simulink model "ACC5v_FFNN_traincgf_30_30_30_ep_50_Nor_20250704"  (R2021a)
settings: Solver=FixedStepAuto  StartTime=0.0  StopTime=T  RelTol=1e-3
undefined symbols (not defined in the file or in its folder): t_gap, Ts, v0_ego, v0_lead, v_set, x0_ego, x0_lead, x_gain, x_offset, y_gain, y_offset
libraries: neural x95
(part 5 of 5)

== system ACC5v_FFNN_traincgf_30_30_30_ep_50_Nor_20250704/Feed-Forward Neural Network/Layer 4/Delays 1 ==
  "p{4}" : Inport  PortDimensions=30
      mask Display: e = 0.06;c1 = [120 230 180]/255;c2 = ([120 230 180]+0)/(256+128);c3 = ([120 230 180]+128)/(256+128);patch([0 1 1 0],[0 0 1 1],c1);patch([0 1 1 1-e 1-e 0+e],[0 0 1 1-e 0+e 0+e],c2);patch([0 0 1 1-e 0+e 0+e],[0 1 1 1-e 1-e 0+e],c3);plot([0 1 1 0 0],[0 0 1 1 0]);
  mux : Mux  Inputs=1
      mask Display: e = 0.06;c1 = [120 150 230]/255;c2 = ([120 150 230]+0)/383;c3 = ([120 150 230]+128)/383;patch([0 1 1 0],[0 0 1 1],c1);patch([0 1 1 1-e 1-e 0+e],[0 0 1 1-e 0+e 0+e],c2);patch([0 0 1 1-e 0+e 0+e],[0 1 1 1-e 1-e 0+e],c3);plot([0 1 1 0 0],[0 0 1 1 0]);disp('Mux')
  "pd{4,3}" : Outport
      mask Display: e = 0.06;c1 = [120 230 180]/255;c2 = ([120 230 180]+0)/(256+128);c3 = ([120 230 180]+128)/(256+128);patch([0 1 1 0],[0 0 1 1],c1);patch([0 1 1 1-e 1-e 0+e],[0 0 1 1-e 0+e 0+e],c2);patch([0 0 1 1-e 0+e 0+e],[0 1 1 1-e 1-e 0+e],c3);plot([0 1 1 0 0],[0 0 1 1 0]);
  wires:
  mux/1 -> "pd{4,3}"/1
  "p{4}"/1 -> mux/1

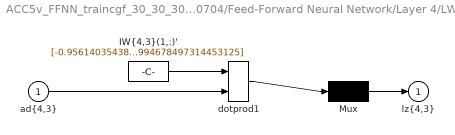
== system ACC5v_FFNN_traincgf_30_30_30_ep_50_Nor_20250704/Feed-Forward Neural Network/Layer 4/LW{4,3} ==
  "ad{4,3}" : Inport  PortDimensions=30
      mask Display: e = 0.06;c1 = [120 230 180]/255;c2 = ([120 230 180]+0)/(256+128);c3 = ([120 230 180]+128)/(256+128);patch([0 1 1 0],[0 0 1 1],c1);patch([0 1 1 1-e 1-e 0+e],[0 0 1 1-e 0+e 0+e],c2);patch([0 0 1 1-e 0+e 0+e],[0 1 1 1-e 1-e 0+e],c3);plot([0 1 1 0 0],[0 0 1 1 0]);
  "IW{4,3}(1,:)'" : Constant  Value=[-0.95614035438404254563238282571546733379364013671875;0.63386249285841611555980534831178374588489532470703125;-0.6415809984175366853520472432137466967105865478515625;-0.66942564451333985697800699199433438479900360107421875;-0.624290829840984162757422382128424942493438720703125;0.38264731629698456316646115737967193126678466796875;-0.582460440130371903677541922661475837230682373046875;-0.358034852656525293124190056914812885224819183349609375;0.5366702941194920750689334454364143311977386474609375;0.0023001892920386790564180046203546226024627685546875;0.797502631479044321594074062886647880077362060546875;-0.8842940174971360978162238097866065800189971923828125;-0.09322973495294946399969404637886327691376209259033203125;0.1445024895044315638159559966879896819591522216796875;0.13013431955435716957936165272258222103118896484375;0.6327509713662682333534803547081537544727325439453125;-0.7246511244316355959682596221682615578174591064453125;-0.39932129407256822251071071150363422930240631103515625;-1.0188460691735048424533260913449339568614959716796875;0.9022147157805451289647180601605214178562164306640625;0.5432291953058989708580384103697724640369415283203125;0.499395785543202908041138243788736872375011444091796875;-0.72227032571813065686683330568484961986541748046875;-0.2933504752943765225836614263243973255157470703125;-0.67495505307956971119409672610345296561717987060546875;-0.0008279921588891206614413409425878853653557598590850830078125;0.62202926737725394712441584488260559737682342529296875;0.27613630396393684662825762643478810787200927734375;0.33668107030330729489975283286185003817081451416015625;0.301005087695761563981733388573047704994678497314453125]
      mask Display: e = 0.06;c1 = [120 150 230]/255;c2 = ([120 150 230]+0)/383;c3 = ([120 150 230]+128)/383;patch([0 1 1 0],[0 0 1 1],c1);patch([0 1 1 1-e 1-e 0+e],[0 0 1 1-e 0+e 0+e],c2);patch([0 0 1 1-e 0+e 0+e],[0 1 1 1-e 1-e 0+e],c3);plot([0 1 1 0 0],[0 0 1 1 0]);disp('weights');
  Mux : Mux  Inputs=1
      mask Display: e = 0.06;c1 = [120 150 230]/255;c2 = ([120 150 230]+0)/383;c3 = ([120 150 230]+128)/383;patch([0 1 1 0],[0 0 1 1],c1);patch([0 1 1 1-e 1-e 0+e],[0 0 1 1-e 0+e 0+e],c2);patch([0 0 1 1-e 0+e 0+e],[0 1 1 1-e 1-e 0+e],c3);plot([0 1 1 0 0],[0 0 1 1 0]);disp('Mux');
  dotprod1 : neural/Weight Functions/dotprod
  "lz{4,3}" : Outport
      mask Display: e = 0.06;c1 = [120 230 180]/255;c2 = ([120 230 180]+0)/(256+128);c3 = ([120 230 180]+128)/(256+128);patch([0 1 1 0],[0 0 1 1],c1);patch([0 1 1 1-e 1-e 0+e],[0 0 1 1-e 0+e 0+e],c2);patch([0 0 1 1-e 0+e 0+e],[0 1 1 1-e 1-e 0+e],c3);plot([0 1 1 0 0],[0 0 1 1 0]);
  wires:
  Mux/1 -> "lz{4,3}"/1
  dotprod1/1 -> Mux/1
  "ad{4,3}"/1 -> dotprod1/2
  "IW{4,3}(1,:)'"/1 -> dotprod1/1
